simulink model "HRTIM"  (R2023b)
settings: Solver=ode3  StartTime=0.0  StopTime=120e-6  RelTol=1e-3
undefined symbols (not defined in the file): HRTIM_SETB1R_REG_VAL, HRTIM_SETB2R_REG_VAL, HRTIM_SETC1R_REG_VAL, HRTIM_SETC2R_REG_VAL, HRTIM_SL
libraries: dspswit3 x8, simulink x6, simulink_extras x4, hdlsllib x4
(part 1 of 2)
settings Model: Creator=Joe  LastModifiedBy=Joe

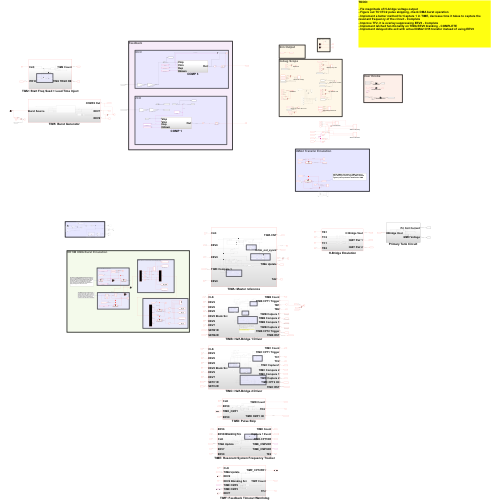
[thumbnail: Simulink's stored preview of the top-level diagram]
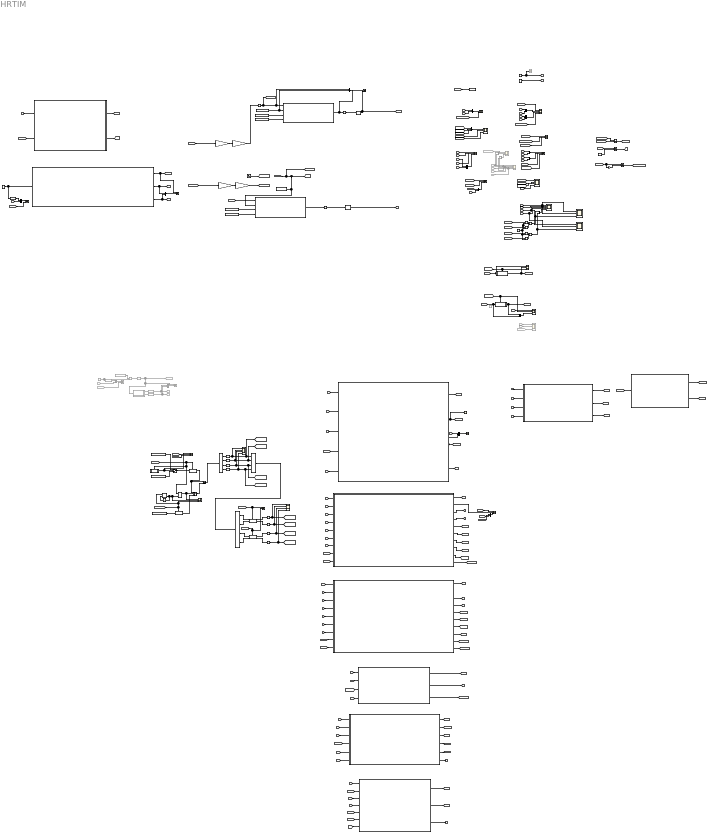
== system HRTIM ==
  note: The DMA2 CH3 trigger is debounced to every 2nd pulse (Hit = 2). This is done so that the output_reset register values can stick for at least 1 resonant cycle, so we are able to witness the pulse skipping waveform at the TB1/2 and TC1/2 outputs
  note: TIMB/C Output 1 and 2 Set Source(s) Shadow Registers
  note: TIMB/C Output 1 and 2 Set Source(s) Active Registers
  note: output_reset DMA Burst Emulation
  note: output_set DMA Burst emulation
  note: Sim Output
  note: ZCD
  note: User Knobs
  note: STM32 System Clocks
  note: Feedback
  note: Debug Scope
  note: HRTIM DMA Burst Emulation
  note: NOTE: DMA2 CH4 write to TIMD Compare 1 goes directly to active register (NOT shadow register) since preload is disabled for TIMD
  note: OCD
  note: TODO:
      |
      | - Fix magnitude of H-bridge voltage output
      | - Figure out TC1/TC2 pulse skipping, check DMA burst operation
      | - Implement a better method for Capture 1 in TIME, decrease time it takes to capture the resonant frequency of the circuit - Complete
      | - Improve TF2, it is overlay suppressing EEV6 - Complete
      | - Implement latched functionality on TIMA EEV9 blanking - COMPLETE
      | - Implement delayed idle exit with actual DMA2 CH5 transfer instead of using EEV9
  note: DMA2 Transfer Emulation
  note: Burst Generator
  note: This seeks to emulate the DMA burst behavior of writing 8 bytes to the HRTIM.BDMADR register when only 4 SFRs are enabled for DMA burst updates (SETB1R,SETB2R, SETC1R and SETC2R). This will update the SFR shadow registers with output_reset[0:3] on 1st DMA2 CH2 trigger, then output_reset[4:7] on 2nd DMA2 CH2. Then resets back to output_reset[0:3] on the 3rd, and on and on.
  APB1 : DiscretePulseGenerator  Period=10  PulseWidth=5  SampleTime=1/(HRTIM_SL.MATLAB.f_discrete)
  APB2 : DiscretePulseGenerator  Period=10  PulseWidth=5  SampleTime=1/(HRTIM_SL.MATLAB.f_discrete)
  COMP 1 : Subsystem
  COMP 3 : Subsystem
  COMP1 : RelationalOperator  Commented=on  Operator=<=  OutDataTypeStr=boolean  RndMeth=Simplest  InputSameDT=off
  COMP3 Hysterisis Lower : Constant  Value=HRTIM_SL.STM32.COMPx_Hdown
  COMP3 Hysterisis Upper : Constant  Value=HRTIM_SL.STM32.COMPx_Hup
  COMP3 INN : Constant  Value=HRTIM_SL.RES_DRV.COMP3.INN
  CT DC Bias : Constant  Value=HRTIM_SL.DRSSTC.vcc/2
  Constant1 : Constant  Value=0  OutDataTypeStr=uint32
  Constant4 : Constant  Commented=on  Value=HRTIM_SL.STM32.VREFINT
  Counter : dspswit3/Counter  Direction=Up  CountEvent=Rising edge  CounterSize=User defined  MaxCount=255  InitialCount=0  Output=Count and Hit  HitValue=HRTIM_SL.MATLAB.output_set_dbnc_cnt  ResetInput=on  SamplesPerFrame=1  Ts=1  CntDtype=double  HitDtype=Boolean
  DMA2 CH1 : Subsystem  TreatAsAtomicUnit=on
  DMA2 CH4 : Subsystem  TreatAsAtomicUnit=on
  Data Type Conversion : DataTypeConversion  OutDataTypeStr=boolean  SaturateOnIntegerOverflow=off  RndMeth=Floor
  Data Type Conversion3 : DataTypeConversion  Commented=on  OutDataTypeStr=boolean  SaturateOnIntegerOverflow=off  RndMeth=Floor
  Data Type Conversion8 : DataTypeConversion  Commented=on  OutDataTypeStr=boolean  SaturateOnIntegerOverflow=off  RndMeth=Floor
  Data Type Conversion9 : DataTypeConversion  Commented=on  OutDataTypeStr=boolean  SaturateOnIntegerOverflow=off  RndMeth=Floor
  Demux : Demux
  Demux1 : Demux
  Disable OCD : Constant  Value=false
  EEV2/6 v FB : Scope  NumInputPorts=2
  FBR : Abs  SaturateOnIntegerOverflow=off
  From1 : From  Commented=on  GotoTag=ZCD_CT_OUT_UNBIASED
  From102 : From  Commented=on  GotoTag=EEV6
  From103 : From  Commented=on  GotoTag=ZCD_CT_OUT
  From20 : From  Commented=on  GotoTag=TB1
  From21 : From  Commented=on  GotoTag=TB2
  From22 : From  Commented=on  GotoTag=TC1
  From23 : From  Commented=on  GotoTag=TC2
  From32 : From  Commented=on  GotoTag=TD2
  From33 : From  Commented=on  GotoTag=EEV8
  From44 : From  Commented=on  GotoTag=DMA2_CH4_TRIGGER
  Goto62 : Goto  Commented=on  GotoTag=EEV7
  Goto63 : Goto  Commented=on  GotoTag=EEV9
  Goto64 : Goto  Commented=on  GotoTag=BURST_SRC
  H-Bridge Emulation : Subsystem
  HBridge v Pri Current v Burst v OCD : Scope  NumInputPorts=3
  HBridge v Txy v FB : Scope  NumInputPorts=4
  HRTIM DMA Burst Op Emulation : Subsystem  TreatAsAtomicUnit=on
  HRTIM DMA Burst Op Emulation1 : Subsystem  TreatAsAtomicUnit=on
  HRTIM EEVx : Scope  NumInputPorts=4
  Half/Full Bridge V OCD Event : Scope  NumInputPorts=4
  Hysterisis Lower : Constant  Value=HRTIM_SL.STM32.COMPx_Hdown
  Hysterisis Upper : Constant  Value=HRTIM_SL.STM32.COMPx_Hup
  Invert ZCD FB : Gain  Gain=-1
  Memory : Memory  Commented=on  InheritSampleTime=on
  Memory2 : Memory  InitialCondition=HRTIM_SETB1R_REG_VAL  InheritSampleTime=on
  Memory3 : Memory  InitialCondition=HRTIM_SETB2R_REG_VAL  InheritSampleTime=on
  Memory4 : Memory  InitialCondition=HRTIM_SETC1R_REG_VAL  InheritSampleTime=on
  Memory5 : Memory  InitialCondition=HRTIM_SETC2R_REG_VAL  InheritSampleTime=on
  Memory6 : Memory  InitialCondition=HRTIM_SETB1R_REG_VAL  InheritSampleTime=on
  Memory7 : Memory  InitialCondition=HRTIM_SETB2R_REG_VAL  InheritSampleTime=on
  Memory8 : Memory  InitialCondition=HRTIM_SETC1R_REG_VAL  InheritSampleTime=on
  Memory9 : Memory  InitialCondition=HRTIM_SETC2R_REG_VAL  InheritSampleTime=on
  Mux{,4,12..13} (4 alike) : Mux  Commented=on  Inputs=2
  Mux{1..3,5..11,14..16,19} (14 alike) : Mux  Inputs=2
  Mux17 : Mux
  Mux18 : Mux  Inputs=3
  OCD Burden Resistor : Gain  Gain=HRTIM_SL.DRSSTC.R_ocd_burden
  OCD CT : Gain  Gain=1/HRTIM_SL.DRSSTC.OCD_CT_N
  OCD Enable/Disable : ManualSwitch
  OR1 : Logic  Operator=OR  IconShape=distinctive  AllPortsSameDT=off  OutDataTypeStr=boolean
  OR3 : Logic  Operator=OR  IconShape=distinctive  AllPortsSameDT=off  OutDataTypeStr=boolean
  Primary Current v Feedback : Scope  NumInputPorts=3
  Primary Tank Circuit : Subsystem
  Pulse Skip Debug : Scope  NumInputPorts=5
  Relational Operator{,1..3} (4 alike) : RelationalOperator  Operator===  OutDataTypeStr=boolean  RndMeth=Simplest  InputSameDT=off
  Rising Edge Of OCB : simulink/Logic and Bit Operations/Detect Rise Positive  vinit=0  OutDataTypeStr=boolean
  Rising Edge Of ZCD FB : simulink/Logic and Bit Operations/Detect Rise Positive  vinit=0  OutDataTypeStr=boolean
  S-R Flip-Flop7 : simulink_extras/Flip Flops/S-R Flip-Flop  initial_condition=0
  SR FF Bypass : ManualSwitch  CurrentSetting=0
  Scope : Scope  Commented=on
  Scope1 : Scope  Commented=on  NumInputPorts=3
  Scope14 : Scope  Commented=on  NumInputPorts=4
  Scope18 : Scope  NumInputPorts=2
  Scope19 : Scope
  Scope2 : Scope  Commented=on  NumInputPorts=2
  Scope20 : Scope
  Scope21 : Scope  NumInputPorts=2
  Scope{3..4,6,23,28,30} (6 alike) : Scope  NumInputPorts=3
  Scope29 : Scope  NumInputPorts=2
  Scope34 : Scope  NumInputPorts=4
  Scope35 : Scope  Commented=on  NumInputPorts=2
  Scope5 : Scope  NumInputPorts=4
  Scope7 : Scope  Commented=on  NumInputPorts=3
  Sum : Sum  Inputs=|++
  Switch1 : Switch  Criteria=u2 ~= 0  SaturateOnIntegerOverflow=off  InputSameDT=off
  Switch2 : Switch  Criteria=u2 ~= 0  SaturateOnIntegerOverflow=off  InputSameDT=off
  TIM2: Start Freq Seed + Lead Time Inject : Subsystem
  TIM5 Burst Gen : DiscretePulseGenerator  Amplitude=HRTIM_SL.DRSSTC.vcc  Period=HRTIM_SL.MATLAB.burst_period_n_samp  PulseWidth=HRTIM_SL.MATLAB.burst_pw_n_samp  PhaseDelay=HRTIM_SL.MATLAB.burst_phase_delay  SampleTime=1/(HRTIM_SL.MATLAB.f_discrete)
  TIM5 Burst Gen1 : DiscretePulseGenerator  Commented=on  Amplitude=HRTIM_SL.DRSSTC.vcc  Period=HRTIM_SL.MATLAB.burst_period_n_samp  PulseWidth=HRTIM_SL.MATLAB.burst_pw_n_samp  SampleTime=1/(HRTIM_SL.MATLAB.f_discrete)
  TIM5: Burst Generator : Subsystem
  TIMA: Master reference : Subsystem
  TIMB Pulse Skip Debug : Scope  NumInputPorts=3
  TIMB: Half-Bridge 1 Driver : Subsystem
  TIMC Pulse Skip Debug : Scope  NumInputPorts=3
  TIMC: Half-Bridge 2 Driver : Subsystem
  TIMD: Pulse Skip : Subsystem
  TIME: Resonant System Frequency Tracker : Subsystem
  TIMF: Feedback Timeout Watchdog : Subsystem
  Tank Circuit v Hbridge : Scope  NumInputPorts=3
  To Workspace : ToWorkspace  VariableName=h_bridge_out  SaveFormat=Timeseries  SampleTime=-1
  Txy v Burst Src v FB : Scope  NumInputPorts=4
  Unit Delay : UnitDelay  SampleTime=-1  HasFrameUpgradeWarning=on
  Update TIMB SETBxR Active Registers : Subsystem  TreatAsAtomicUnit=on
  Update TIMB SETCxR Active Registers : Subsystem  TreatAsAtomicUnit=on
  ZCD Burden Resistor : Gain  Gain=HRTIM_SL.DRSSTC.R_zcd_burden
  ZCD CT : Gain  Gain=1/HRTIM_SL.DRSSTC.ZCD_CT_N
  ZCD Current Feedback : Sin  Amplitude=HRTIM_SL.DRSSTC.vcc/2  Frequency=(HRTIM_SL.DRSSTC.f_pri_res*HRTIM_SL.DRSSTC.f_fb_skew)*2*pi  SampleTime=0
  ZCD FB Select : ManualSwitch  CurrentSetting=0
  ZCD Invert FB Select : ManualSwitch  CurrentSetting=0
  Zero-Order Hold : ZeroOrderHold  SampleTime=1/(HRTIM_SL.MATLAB.f_discrete)
  Zero-Order Hold2 : ZeroOrderHold  SampleTime=1/(HRTIM_SL.MATLAB.f_discrete)
  Zero-Order Hold3 : ZeroOrderHold  Commented=on  SampleTime=1/(HRTIM_SL.MATLAB.f_discrete)
  gen_eev7_eev1 : MATLAB Function  Commented=on  TreatAsAtomicUnit=on
  out_reset_toggle : Subsystem  TreatAsAtomicUnit=on
  output_reset[0:3] : Constant  Value=HRTIM_SL.RES_DRV.output_reset03
  output_reset[4:7] : Constant  Value=HRTIM_SL.RES_DRV.output_reset47
  output_set : Constant  Value=HRTIM_SL.RES_DRV.output_set
  wires:
  Sum/1 -> [ZCD_CT_OUT]  "Biased CT Out"
  CT DC Bias/1 -> COMP 1/2(Vinn), Sum/2  "CT DC Bias"
  Zero-Order Hold/1 -> Rising Edge Of ZCD FB/1  "EEV6"
  APB2/1 -> Scope/1, [APB2]  "APB2"
  APB1/1 -> [APB1]  "APB1"
  From20/1 -> Scope14/1, Mux/1  "TB1"
  From21/1 -> Mux/2, Scope14/2  "TB2"
  From22/1 -> Mux4/1, Scope14/3  "TC1"
  From23/1 -> Mux4/2, Scope14/4  "TC2"
  [ZCD_CT_OUT] -> Scope18/2  "ZCD CT Out"
  [EEV6] -> Mux1/2  "EEV6"
  Mux1/1 -> Scope18/1
  TIM5 Burst Gen/1 -> TIM5: Burst Generator/1(Burst Source), Data Type Conversion/1  "Burst Source"
  Data Type Conversion/1 -> Mux1/1  "Burst Source"
  FBR/1 -> [OCD_FB_RECTIFIED], COMP 3/1(Vinp), Mux2/1  "OCD CT Out Rectified"
  COMP 3/1(Out) -> Zero-Order Hold2/1, Scope23/2  "COMP3 Out"
  DMA2 CH4/1(Out1) -> Mux3/1, [TIMD_CMP1DR]  "TIMD Compare 1"
  [DMA2_CH4_TRIGGER] -> DMA2 CH4/Trigger, Scope28/2  "DMA2 CH4 Trigger"
  [TIME_CNT] -> Scope28/1  "TIME Count"
  Mux3/1 -> Scope28/3
  [DMA2_CH1_TRIGGER] -> DMA2 CH1/Trigger, Scope30/3  "DMA2 CH1 Trigger"
  [TIME_CPT1ER] -> Scope30/1, DMA2 CH1/1(In1)  "TIME Capture 1"
  [APB2] -> TIMD: Pulse Skip/1(CLK)
  [EEV8] -> TIMD: Pulse Skip/2(EEV8)
  [TIMD_CMP1DR] -> TIMD: Pulse Skip/3(TIMD_CMP1)
  [EEV9] -> TIMD: Pulse Skip/4(EEV9)
  TIMD: Pulse Skip/1(TIMD Count) -> [TIMD_CNT]
  TIMD: Pulse Skip/2(TD2) -> [TD2]
  [APB2] -> TIMF: Feedback Timeout Watchdog/1(CLK)
  [TIMA_UPDATE] -> TIMF: Feedback Timeout Watchdog/2(TIMA Update)  "TIMA Update"
  [EEV2] -> TIMF: Feedback Timeout Watchdog/3(EEV2)
  [TE2] -> TIMF: Feedback Timeout Watchdog/4(EEV2 Blanking Src)
  [TIME_CMP2ER] -> TIMF: Feedback Timeout Watchdog/5(TIME CMP2)  "TIME CMP2"
  [TIME_CMP3ER] -> TIMF: Feedback Timeout Watchdog/6(TIME CMP3)  "TIME CMP3"
  [EEV7] -> TIMF: Feedback Timeout Watchdog/7(EEV7)
  TIMF: Feedback Timeout Watchdog/1(TIMF_CPT2FR1) -> [TIMF_CPT2FR1]
  TIMF: Feedback Timeout Watchdog/2(TIMF Count) -> [TIMF_CNT]
  TIMF: Feedback Timeout Watchdog/3(TF2) -> [TF2]
  [EEV6] -> TIME: Resonant System Frequency Tracker/1(EEV6)  "EEV6"
  [TF2] -> TIME: Resonant System Frequency Tracker/2(EEV6 Blanking Src)  "TF2"
  [APB2] -> TIME: Resonant System Frequency Tracker/3(CLK)
  [TIMA_UPDATE] -> TIME: Resonant System Frequency Tracker/4(TIMA Update)  "TIMA Update"
  [EEV7] -> TIME: Resonant System Frequency Tracker/5(EEV7)  "EEV7"
  [EEV9] -> TIME: Resonant System Frequency Tracker/6(EEV9)  "EEV9"
  TIME: Resonant System Frequency Tracker/1(TIME Count) -> [TIME_CNT]
  TIME: Resonant System Frequency Tracker/2(Capture 1 Event) -> [DMA2_CH1_TRIGGER]
  TIME: Resonant System Frequency Tracker/3(TIME.CPT1ER) -> [TIME_CPT1ER]
  TIME: Resonant System Frequency Tracker/4(TIME_CMP2ER) -> [TIME_CMP2ER]
  TIME: Resonant System Frequency Tracker/5(TIME_CMP3ER) -> [TIME_CMP3ER]
  TIME: Resonant System Frequency Tracker/6(TE2) -> [TE2]
  From1/1 -> Scope1/1
  Mux/1 -> Scope1/2
  Mux4/1 -> Scope1/3
  [TIMB_CNT] -> Scope4/1  "TIMB CNT"
  Mux5/1 -> Scope4/3
  [TIMB_CPT1BR] -> Mux5/1  "Capture 1 Reg"
  [TIMB_CMP2BR] -> Mux5/2  "Compare 2 Reg"
  Rising Edge Of ZCD FB/1 -> [EEV6]  "EEV6 RE"
  [EEV9] -> Mux6/2  "EEV9 (BURST RE)"
  [EEV7] -> Mux6/1  "EEV7(BURST LL)"
  [EEV2] -> HRTIM EEVx/1  "EEV2 (TRGO RE)"
  [EEV6] -> HRTIM EEVx/2  "EEV6 (ZCD RE)"
  [EEV8] -> HRTIM EEVx/3  "EEV8 (OCD RE)"
  Mux6/1 -> HRTIM EEVx/4
  [APB2] -> TIMB: Half-Bridge 1 Driver/1(CLK)
  [EEV2] -> TIMB: Half-Bridge 1 Driver/2(EEV2)  "EEV2"
  [EEV6] -> TIMB: Half-Bridge 1 Driver/3(EEV6)  "EEV6"
  TIMB: Half-Bridge 1 Driver/1(TIMB Count) -> [TIMB_CNT]
  TIMB: Half-Bridge 1 Driver/2(TIMB CPT1 Trigger) -> Scope4/2
  TIMB: Half-Bridge 1 Driver/3(TB1) -> [TB1]
  TIMB: Half-Bridge 1 Driver/4(TB2) -> [TB2]
  TIMB: Half-Bridge 1 Driver/7(TIMB Compare 1) -> [TIMB_CMP1BR]
  TIMB: Half-Bridge 1 Driver/6(TIMB Compare 2) -> [TIMB_CMP2BR]
  TIMB: Half-Bridge 1 Driver/5(TIMB Catpure 1) -> [TIMB_CPT1BR]
  TIMC: Half-Bridge 2 Driver/5(TIMC Capture1) -> [TIMC_CPT1BR]
  TIMC: Half-Bridge 2 Driver/6(TIMC Compare 2) -> [TIMC_CMP2BR]
  TIMC: Half-Bridge 2 Driver/8(TIMC Capture 2) -> [TIMC_CPT2CR]  "TIMC CPT2 eg"
  TIMC: Half-Bridge 2 Driver/7(TIMC Compare 1) -> [TIMC_CMP1CR]
  TIMC: Half-Bridge 2 Driver/4(TC2) -> [TC2]
  TIMC: Half-Bridge 2 Driver/3(TC1) -> [TC1]
  TIMC: Half-Bridge 2 Driver/1(TIMC Count) -> [TIMC_CNT]
  [APB2] -> TIMC: Half-Bridge 2 Driver/1(CLK)
  [EEV2] -> TIMC: Half-Bridge 2 Driver/2(EEV2)
  [EEV6] -> TIMC: Half-Bridge 2 Driver/3(EEV6)
  [EEV8] -> TIMC: Half-Bridge 2 Driver/4(EEV8)
  [TD2] -> TIMC: Half-Bridge 2 Driver/5(EEV8 Blank Src)
  TIMC: Half-Bridge 2 Driver/9(TIMC CPT2 Hit) -> [DMA2_CH4_TRIGGER]  "TIMC CPT2 Hit"
  Rising Edge Of OCB/1 -> [EEV8_RE], Scope23/3  "EEV8 RE"
  TIMB: Half-Bridge 1 Driver/8(TIMB Capture 2) -> [TIMB_CPT2BR]
  TIMB: Half-Bridge 1 Driver/9(TIMB CPT2 Trigger) -> [DMA2_CH2_TRIGGER]  "TIMB CPT2 Trigger"
  [EEV8] -> TIMB: Half-Bridge 1 Driver/4(EEV8)  "EEV8"
  [TA2] -> TIMB: Half-Bridge 1 Driver/5(EEV8 Blank Src)
  [APB2] -> TIMA: Master reference/1(CLK)
  [EEV6] -> TIMA: Master reference/2(EEV6)  "EEV6"
  [EEV9] -> TIMA: Master reference/3(EEV9)  "EEV9"
  [TIMD_CMP1DR] -> TIMA: Master reference/4(TIMD Compare 1)  "TIMD Compare 1"
  [EEV8] -> TIMA: Master reference/5(EEV8)  "EEV8"
  TIMA: Master reference/1(TIMA CNT) -> [TIMA_CNT]
  TIMA: Master reference/2(hrtim_out_sync2) -> Scope19/1, [hrtim_out_sync2]  "hrtim_out_sync2"
  TIMA: Master reference/3(TIMA Update) -> Mux7/2, [TIMA_UPDATE]  "TIMA Update"
  TIMA: Master reference/4(TA2) -> [TA2]
  Mux7/1 -> Scope20/1
  [EEV6] -> Mux7/1
  Mux8/1 -> Scope21/2
  [EEV7] -> TIMB: Half-Bridge 1 Driver/7(EEV7)
  [EEV9] -> TIMB: Half-Bridge 1 Driver/6(EEV9)
  [TB1] -> Mux10/1  "TB1"
  [TB2] -> Mux10/2  "TB2"
  [TC2] -> Mux11/2  "TC2"
  [TC1] -> Mux11/1  "TC1"
  Mux10/1 -> Txy v Burst Src v FB/1
  Mux11/1 -> Txy v Burst Src v FB/2
  [BURST_SRC] -> Txy v Burst Src v FB/3  "Burst Src"
  [ZCD_CT_OUT_UNBIASED] -> Txy v Burst Src v FB/4  "ZCD"
  [EEV7] -> TIMC: Half-Bridge 2 Driver/7(EEV7)
  [EEV9] -> TIMC: Half-Bridge 2 Driver/6(EEV9)
  Switch1/1 -> HRTIM DMA Burst Op Emulation/1(In1)
  [DMA2_CH2_TRIGGER] -> out_reset_toggle/Trigger, S-R Flip-Flop7/1, HRTIM DMA Burst Op Emulation/Trigger  "TIMB Capture 2"
  output_reset[0:3]/1 -> Switch1/1
  output_reset[4:7]/1 -> Switch1/3
  Demux/3 -> Memory8/1
  Demux/4 -> Memory9/1
  HRTIM DMA Burst Op Emulation/1(Out1) -> SR FF Bypass/1, Switch2/1  "SETxyR Shadow Registers"
  ZCD CT/1 -> ZCD Burden Resistor/1
  [ZCD_FB_SRC] -> [ZCD_CT_OUT_UNBIASED], Sum/1  "ZCD Out"
  DMA2 CH1/1(Out1) -> Scope30/2, [TIM2_ARR_SH]  "TIM2 ARR Shadow Register"
  [ZCD_CT_OUT] -> COMP 1/1(Vinp)  "Vinp"
  Hysterisis Upper/1 -> COMP 1/3(Hup)  "Hup"
  Hysterisis Lower/1 -> COMP 1/4(Hdown)  "Hdown"
  COMP 1/1(Out) -> Zero-Order Hold/1  "COMP1 Out"
  ZCD Burden Resistor/1 -> [ZCD_FB_SRC_SAMPLED]  "Sampled Feedback"
  ZCD Current Feedback/1 -> [ZCD_FB_SRC_GENERATED]  "Generated Feedback"
  ZCD FB Select/1 -> [ZCD_FB_SRC]  "ZCD Out"
  [ZCD_FB_SRC_GENERATED] -> ZCD FB Select/1
  [ZCD_FB_SRC_SAMPLED] -> ZCD FB Select/2
  COMP3 Hysterisis Upper/1 -> COMP 3/3(Hup)  "Hup"
  COMP3 Hysterisis Lower/1 -> COMP 3/4(Hdown)  "Hdown"
  COMP3 INN/1 -> Mux2/2, COMP 3/2(Vinn)  "COMP3 INN"
  Zero-Order Hold2/1 -> Rising Edge Of OCB/1  "EEV8"
  Mux2/1 -> Scope23/1
  OCD CT/1 -> OCD Burden Resistor/1
  OCD Burden Resistor/1 -> FBR/1  "Sampled Feedback"
  [HBRIDGE_OUT] -> To Workspace/1
  Disable OCD/1 -> OCD Enable/Disable/2
  OCD Enable/Disable/1 -> [EEV8]  "EEV8"
  [EEV8_RE] -> OCD Enable/Disable/1  "EEV8 Rising Edge"
  [PRI_CURRENT] -> Primary Current v Feedback/1  "Primary Current"
  [ZCD_CT_OUT_UNBIASED] -> Primary Current v Feedback/2  "ZCD FB"
  [OCD_FB_RECTIFIED] -> Primary Current v Feedback/3  "OCD FB RECT"
  [TB2] -> Mux14/2  "TB2"
  [TC2] -> Mux15/2  "TC2"
  Mux15/1 -> HBridge v Txy v FB/3
  [TC1] -> Mux15/1  "TC1"
  [TB1] -> Mux14/1  "TB1"
  Mux14/1 -> HBridge v Txy v FB/2
  [ZCD_CT_OUT_UNBIASED] -> HBridge v Txy v FB/4  "ZCD"
  [HBRIDGE_OUT] -> HBridge v Txy v FB/1  "H Bridge Out"
  [TIME_CPT1ER] -> DMA2 CH4/1(In1), Mux3/2  "TIME Capture 1"
  gen_eev7_eev1/2(eev9) -> Data Type Conversion9/1
  Data Type Conversion9/1 -> Goto63/1, Mux13/2  "EEV9"
  Mux13/1 -> Scope35/2
  Zero-Order Hold3/1 -> Goto64/1, gen_eev7_eev1/1(comp4_out), Scope35/1  "COMP4 Out"
  From102/1 -> Mux12/2  "EEV6"
  Constant4/1 -> COMP1/1
  gen_eev7_eev1/1(eev7) -> Data Type Conversion8/1
  Mux12/1 -> Scope2/1
  Data Type Conversion8/1 -> Mux13/1, Goto62/1  "EEV7"
  Data Type Conversion3/1 -> Mux12/1  "Burst Source"
  TIM5 Burst Gen1/1 -> Data Type Conversion3/1, COMP1/2  "Burst Source"
  COMP1/1 -> Zero-Order Hold3/1
  From103/1 -> Scope2/2  "ZCD CT Out"
  [EEV2] -> Mux16/1  "EEV2 (TRGO RE)"
  [EEV6] -> Mux16/2  "EEV6 (ZCD RE)"
  Mux16/1 -> EEV2/6 v FB/1
  [ZCD_CT_OUT_UNBIASED] -> EEV2/6 v FB/2  "ZCD"
  [ZCD_PRI_CURRENT] -> ZCD CT/1
  [PRI_CURRENT] -> ZCD Invert FB Select/1, Invert ZCD FB/1  "Primary Current"
  Invert ZCD FB/1 -> ZCD Invert FB Select/2
  [PRI_CURRENT] -> OCD CT/1  "Primary Current"
  ZCD Invert FB Select/1 -> [ZCD_PRI_CURRENT]  "To ZCD Feedback Circuit"
  [PRI_CURRENT] -> Tank Circuit v Hbridge/2  "Pri Current"
  [MMC_Voltage] -> Tank Circuit v Hbridge/3  "MMC Voltage"
  [IGBT_PAIR1] -> Mux18/1  "IGBT Pair1"
  Mux18/1 -> Tank Circuit v Hbridge/1
  [IGBT_PAIR2] -> Mux18/2  "IGBT Pair2"
  [HBRIDGE_OUT] -> Mux18/3  "Hbridge Out"
  [APB1] -> TIM2: Start Freq Seed + Lead Time Inject/1(CLK)  "APB1"
  [hrtim_out_sync2] -> TIM2: Start Freq Seed + Lead Time Inject/2(ITR10)  "ITR10"
  TIM2: Start Freq Seed + Lead Time Inject/1(TIM2 Count) -> [TIM2_CNT]  "TIM2 CNT"
  TIM2: Start Freq Seed + Lead Time Inject/2(TIM2 TRGO RE) -> [EEV2]  "TIM2 TRGO RE"
  out_reset_toggle/1(Out1) -> Scope6/1, Switch1/2  "out_reset_toggle"
  Demux1/1 -> Update TIMB SETBxR Active Registers/1(In1)  "SETB1R SH"
  Update TIMB SETBxR Active Registers/1(Out1) -> Memory2/1
  Demux1/2 -> Update TIMB SETBxR Active Registers/2(In2)  "SETB2R SH"
  Update TIMB SETBxR Active Registers/2(Out2) -> Memory3/1  "SETB2R Active"
  [TIMB_UPDATE_TRIG] -> Scope29/1, Update TIMB SETBxR Active Registers/Trigger  "TIMB Update Trigger"
  Demux1/3 -> Update TIMB SETCxR Active Registers/1(In1)  "SETC1R SH"
  Demux1/4 -> Update TIMB SETCxR Active Registers/2(In2)  "SETC2R SH"
  Update TIMB SETCxR Active Registers/1(Out1) -> Memory4/1  "SETC1R Active"
  Update TIMB SETCxR Active Registers/2(Out2) -> Memory5/1  "SETC2R Active"
  [TIMC_UPDATE_TRIG] -> Scope29/2, Update TIMB SETCxR Active Registers/Trigger  "TIMC Update Trigger"
  TIMB: Half-Bridge 1 Driver/10(TIMB RST) -> [TIMB_UPDATE_TRIG]  "TIMB RST Triggers Update"
  TIMC: Half-Bridge 2 Driver/10(TIMC RST) -> [TIMC_UPDATE_TRIG]  "TIMC RST Triggers Update"
  [TIMB_SETB1R] -> TIMB: Half-Bridge 1 Driver/8(SETB1R)
  [TIMB_SETB2R] -> TIMB: Half-Bridge 1 Driver/9(SETB2R)
  [TIMC_SETC2R] -> TIMC: Half-Bridge 2 Driver/9(SETC2R)
  [TIMC_SETC1R] -> TIMC: Half-Bridge 2 Driver/8(SETC1R)
  Memory2/1 -> [TIMB_SETB1R], Scope34/1
  Memory3/1 -> [TIMB_SETB2R], Scope34/2
  Memory4/1 -> Scope34/3, [TIMC_SETC1R]
  Memory5/1 -> Scope34/4, [TIMC_SETC2R]
  Memory6/1 -> Mux17/1, [TIMB_SETB1R_SH], Scope5/1  "SETB1R SH"
  Memory7/1 -> Mux17/2, [TIMB_SETB2R_SH], Scope5/2  "SETB2R SH"
  Memory8/1 -> [TIMC_SETC1R_SH], Mux17/3, Scope5/3  "SETC1R SH"
  Memory9/1 -> [TIMC_SETC2R_SH], Mux17/4, Scope5/4  "SETC2R SH"
  Demux/1 -> Memory6/1
  Demux/2 -> Memory7/1
  Mux17/1 -> Demux1/1
  [BURST_SRC] -> Mux19/1  "Burst Src"
  [EEV8] -> Mux19/2  "EEV8"
  [HBRIDGE_OUT] -> HBridge v Pri Current v Burst v OCD/1  "Hbridge Out"
  [PRI_CURRENT] -> HBridge v Pri Current v Burst v OCD/2  "Pri Current"
  Mux19/1 -> HBridge v Pri Current v Burst v OCD/3
  TIMD: Pulse Skip/3("TIMD CMP1 Hit ") -> [DMA2_CH3_TRIGGER]  "TIMD CMP1 Hit"
  output_set/1 -> HRTIM DMA Burst Op Emulation1/1(In1)
  S-R Flip-Flop7/1 -> Switch2/2, Scope3/1  "Q"
  [DMA2_CH3_TRIGGER] -> Scope3/3, Counter/1, HRTIM DMA Burst Op Emulation1/Trigger  "TIMD Compare 1"
  HRTIM DMA Burst Op Emulation1/1(Out1) -> Switch2/3
  SR FF Bypass/1 -> Demux/1
  Switch2/1 -> SR FF Bypass/2
  Counter/2 -> S-R Flip-Flop7/2, Scope3/2, Unit Delay/1  "SR FF Reset"
  Unit Delay/1 -> Counter/2
  TIM5: Burst Generator/3(EEV9) -> [EEV9], Mux8/2  "EEV9"
  TIM5: Burst Generator/2(EEV7) -> Mux8/1, [EEV7]  "EEV7"
  TIM5: Burst Generator/1(COMP4 Out) -> Scope21/1, [BURST_SRC]
  Relational Operator/1 -> OR3/1
  [TIMB_SETB1R] -> Relational Operator/1
  Relational Operator1/1 -> OR3/2
  Constant1/1 -> Relational Operator1/2, Relational Operator/2, Relational Operator2/2, Relational Operator3/2
  [TIMB_SETB2R] -> Relational Operator1/1
  [TIMC_SETC2R] -> Relational Operator3/1
  Relational Operator2/1 -> OR1/1
  Relational Operator3/1 -> OR1/2
  [TIMC_SETC1R] -> Relational Operator2/1
  [TB1] -> Pulse Skip Debug/1, TIMB Pulse Skip Debug/1  "TB1"
  [TB2] -> Pulse Skip Debug/2, TIMB Pulse Skip Debug/2  "TB2"
  [TC1] -> TIMC Pulse Skip Debug/1, Pulse Skip Debug/3  "TC1"
  OR3/1 -> Mux9/1, TIMB Pulse Skip Debug/3  "TIMB SET Disabled"
  OR1/1 -> TIMC Pulse Skip Debug/3, Mux9/2  "TIMC SET Disabled"
  [TC2] -> Pulse Skip Debug/4, TIMC Pulse Skip Debug/2  "TC2"
  Mux9/1 -> Pulse Skip Debug/5
  [TIMB_UPDATE_TRIG] -> Scope6/2  "TIMB Update Trigger"
  [TIMC_UPDATE_TRIG] -> Scope6/3  "TIMC Update Trigger"
  From32/1 -> Scope7/1  "TD2"
  From33/1 -> Scope7/2  "EEV8"
  From44/1 -> Scope7/3  "DMA2 CH4 Trigger"
  [IGBT_PAIR1] -> Half/Full Bridge V OCD Event/1  "Half Bridge 1"
  [EEV8] -> Half/Full Bridge V OCD Event/4  "EEV8 (OCD)"
  [HBRIDGE_OUT] -> Half/Full Bridge V OCD Event/3  "Full Bridge"
  [IGBT_PAIR2] -> Half/Full Bridge V OCD Event/2  "Half Bridge 2"
  [TB1] -> H-Bridge Emulation/1(TB1)  "TB1"
  [TC2] -> H-Bridge Emulation/2(TC2)  "TC2"
  [TC1] -> H-Bridge Emulation/3(TC1)  "TC1"
  [TB2] -> H-Bridge Emulation/4(TB2)  "TB2"
  H-Bridge Emulation/1(H Bridge Vout) -> [HBRIDGE_OUT]  "Full Bridge Out"
  H-Bridge Emulation/2(IGBT Pair 1) -> [IGBT_PAIR1]  "Half Bridge 1 Out"
  H-Bridge Emulation/3(IGBT Pair 2) -> [IGBT_PAIR2]  "Half Bridge 2 Out"
  [HBRIDGE_OUT] -> Primary Tank Circuit/1(HBridge Vout)  "HBridge Vout"
  Primary Tank Circuit/1(Pri Coil Current) -> [PRI_CURRENT]  "Primary Current"
  Primary Tank Circuit/2(MMC Voltage) -> [MMC_Voltage]  "MMC Voltage"

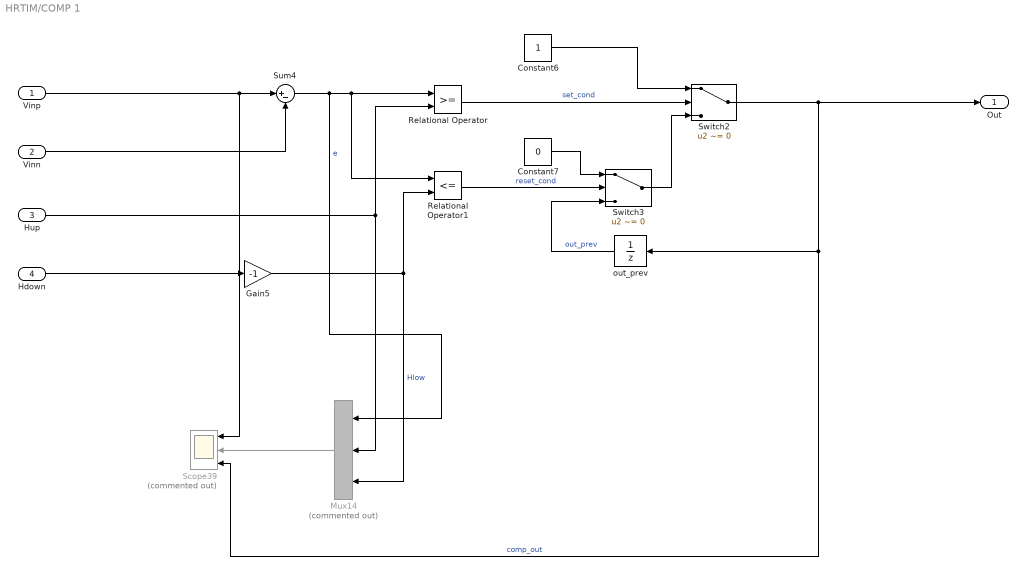
== system HRTIM/COMP 1 ==
  Vinp : Inport
  Vinn : Inport  Port=2
  Hup : Inport  Port=3
  Hdown : Inport  Port=4
  Constant6 : Constant
  Constant7 : Constant  Value=0
  Gain5 : Gain  Gain=-1
  Mux14 : Mux  Commented=on  Inputs=3
  Relational Operator : RelationalOperator  OutDataTypeStr=boolean  RndMeth=Simplest  InputSameDT=off
  Relational Operator1 : RelationalOperator  Operator=<=  OutDataTypeStr=boolean  RndMeth=Simplest  InputSameDT=off
  Scope39 : Scope  Commented=on  NumInputPorts=3
  Sum4 : Sum  Inputs=|+-
  Switch2 : Switch  Criteria=u2 ~= 0  SaturateOnIntegerOverflow=off  InputSameDT=off
  Switch3 : Switch  Criteria=u2 ~= 0  SaturateOnIntegerOverflow=off  InputSameDT=off
  out_prev : UnitDelay  SampleTime=-1  HasFrameUpgradeWarning=on
  Out : Outport
  wires:
  Sum4/1 -> Mux14/1, Relational Operator/1, Relational Operator1/1  "e"
  Relational Operator/1 -> Switch2/2  "set_cond"
  Switch2/1 -> Out/1, out_prev/1, Scope39/3  "comp_out"
  Relational Operator1/1 -> Switch3/2  "reset_cond"
  Mux14/1 -> Scope39/2
  Vinn/1 -> Sum4/2
  Gain5/1 -> Mux14/3, Relational Operator1/2  "Hlow"
  Constant6/1 -> Switch2/1
  out_prev/1 -> Switch3/3  "out_prev"
  Hup/1 -> Mux14/2, Relational Operator/2
  Constant7/1 -> Switch3/1
  Vinp/1 -> Scope39/1, Sum4/1
  Switch3/1 -> Switch2/3
  Hdown/1 -> Gain5/1

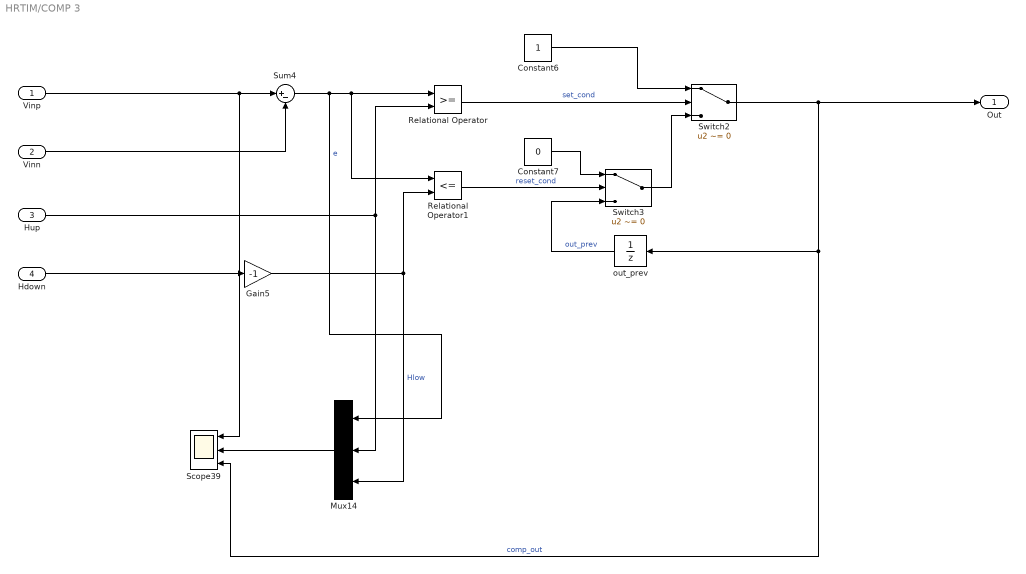
== system HRTIM/COMP 3 ==
  Vinp : Inport
  Vinn : Inport  Port=2
  Hup : Inport  Port=3
  Hdown : Inport  Port=4
  Constant6 : Constant
  Constant7 : Constant  Value=0
  Gain5 : Gain  Gain=-1
  Mux14 : Mux  Inputs=3
  Relational Operator : RelationalOperator  OutDataTypeStr=boolean  RndMeth=Simplest  InputSameDT=off
  Relational Operator1 : RelationalOperator  Operator=<=  OutDataTypeStr=boolean  RndMeth=Simplest  InputSameDT=off
  Scope39 : Scope  NumInputPorts=3
  Sum4 : Sum  Inputs=|+-
  Switch2 : Switch  Criteria=u2 ~= 0  SaturateOnIntegerOverflow=off  InputSameDT=off
  Switch3 : Switch  Criteria=u2 ~= 0  SaturateOnIntegerOverflow=off  InputSameDT=off
  out_prev : UnitDelay  SampleTime=-1  HasFrameUpgradeWarning=on
  Out : Outport
  wires:
  Sum4/1 -> Mux14/1, Relational Operator/1, Relational Operator1/1  "e"
  Relational Operator/1 -> Switch2/2  "set_cond"
  Switch2/1 -> Out/1, out_prev/1, Scope39/3  "comp_out"
  Relational Operator1/1 -> Switch3/2  "reset_cond"
  Mux14/1 -> Scope39/2
  Vinn/1 -> Sum4/2
  Gain5/1 -> Mux14/3, Relational Operator1/2  "Hlow"
  Constant6/1 -> Switch2/1
  out_prev/1 -> Switch3/3  "out_prev"
  Hup/1 -> Mux14/2, Relational Operator/2
  Constant7/1 -> Switch3/1
  Vinp/1 -> Scope39/1, Sum4/1
  Switch3/1 -> Switch2/3
  Hdown/1 -> Gain5/1

== system HRTIM/DMA2 CH1 ==
  In1 : Inport
  Trigger : TriggerPort  VariantControl=(inherit)
  Out1 : Outport
  wires:
  In1/1 -> Out1/1

== system HRTIM/DMA2 CH4 ==
  In1 : Inport
  Trigger : TriggerPort  VariantControl=(inherit)
  Out1 : Outport
  wires:
  In1/1 -> Out1/1

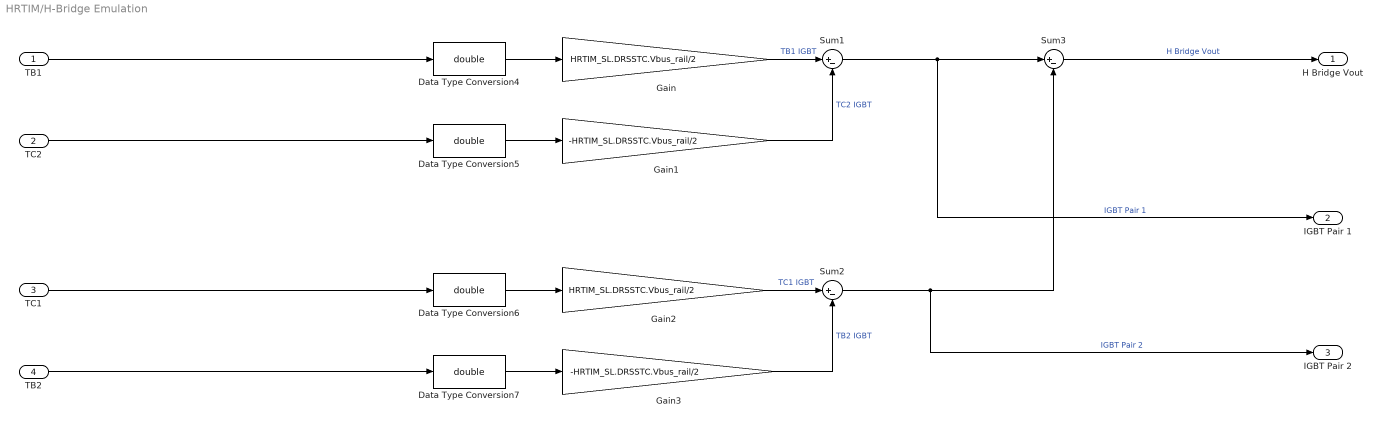
== system HRTIM/H-Bridge Emulation ==
  TB1 : Inport
  TC2 : Inport  Port=2
  TC1 : Inport  Port=3
  TB2 : Inport  Port=4
  Data Type Conversion{4..7} (4 alike) : DataTypeConversion  OutDataTypeStr=double  SaturateOnIntegerOverflow=off  RndMeth=Floor
  Gain : Gain  Gain=HRTIM_SL.DRSSTC.Vbus_rail/2
  Gain1 : Gain  Gain=-HRTIM_SL.DRSSTC.Vbus_rail/2
  Gain2 : Gain  Gain=HRTIM_SL.DRSSTC.Vbus_rail/2
  Gain3 : Gain  Gain=-HRTIM_SL.DRSSTC.Vbus_rail/2
  Sum1 : Sum  Inputs=|+-
  Sum2 : Sum  Inputs=|+-
  Sum3 : Sum  Inputs=|+-
  H Bridge Vout : Outport
  IGBT Pair 1 : Outport  Port=2
  IGBT Pair 2 : Outport  Port=3
  wires:
  Gain2/1 -> Sum2/1  "TC1 IGBT"
  Sum1/1 -> IGBT Pair 1/1, Sum3/1  "IGBT Pair 1"
  Data Type Conversion7/1 -> Gain3/1
  Gain1/1 -> Sum1/2  "TC2 IGBT"
  Data Type Conversion4/1 -> Gain/1
  Sum2/1 -> IGBT Pair 2/1, Sum3/2  "IGBT Pair 2"
  Data Type Conversion6/1 -> Gain2/1
  Gain3/1 -> Sum2/2  "TB2 IGBT"
  Gain/1 -> Sum1/1  "TB1 IGBT"
  Data Type Conversion5/1 -> Gain1/1
  TB1/1 -> Data Type Conversion4/1
  TC1/1 -> Data Type Conversion6/1
  Sum3/1 -> H Bridge Vout/1  "H Bridge Vout"
  TB2/1 -> Data Type Conversion7/1
  TC2/1 -> Data Type Conversion5/1

== system HRTIM/HRTIM DMA Burst Op Emulation ==
  In1 : Inport
  Trigger : TriggerPort  VariantControl=(inherit)
  Out1 : Outport  InitialOutput=HRTIM_SL.RES_DRV.output_set
  wires:
  In1/1 -> Out1/1

== system HRTIM/HRTIM DMA Burst Op Emulation1 ==
  In1 : Inport
  Trigger : TriggerPort  VariantControl=(inherit)
  Out1 : Outport  InitialOutput=HRTIM_SL.RES_DRV.output_set
  wires:
  In1/1 -> Out1/1

== system HRTIM/Primary Tank Circuit ==
  HBridge Vout : Inport
  Demux2 : Demux  Outputs=2
  Primary Tank Circuit : StateSpace  A=HRTIM_SL.MATLAB.PRI_TANK.A  B=HRTIM_SL.MATLAB.PRI_TANK.B  C=HRTIM_SL.MATLAB.PRI_TANK.C  D=HRTIM_SL.MATLAB.PRI_TANK.D  InitialCondition=HRTIM_SL.MATLAB.PRI_TANK.x0
  Scope36 : Scope  Commented=on  NumInputPorts=3
  Pri Coil Current : Outport
  MMC Voltage : Outport  Port=2
  wires:
  Demux2/1 -> Pri Coil Current/1, Scope36/2  "Pri Coil Current"
  HBridge Vout/1 -> Primary Tank Circuit/1, Scope36/1
  Primary Tank Circuit/1 -> Demux2/1
  Demux2/2 -> MMC Voltage/1, Scope36/3  "MMC Voltage"

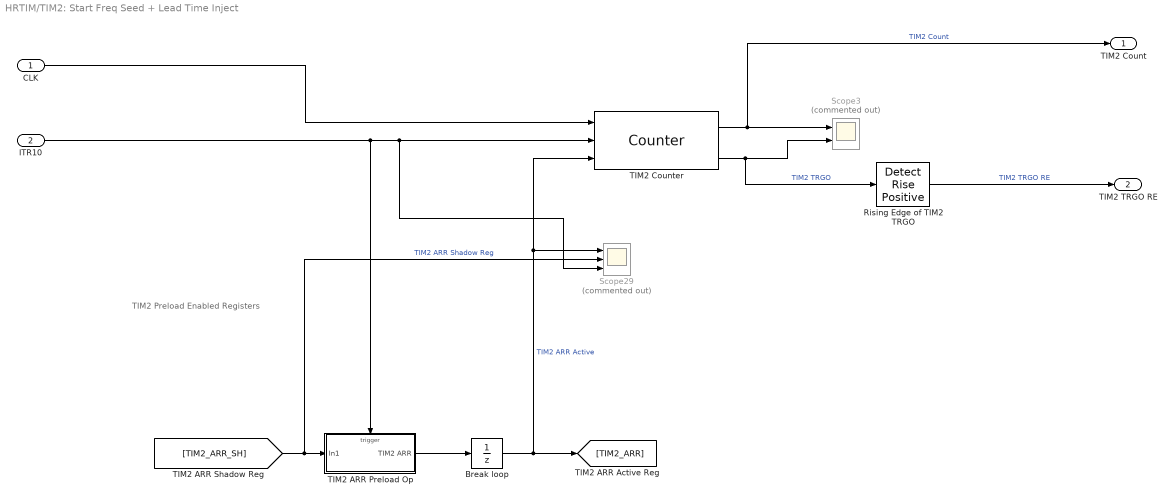
== system HRTIM/TIM2: Start Freq Seed + Lead Time Inject ==
  note: TIM2 Preload Enabled Registers
  CLK : Inport
  ITR10 : Inport  Port=2
  Break loop : UnitDelay  InitialCondition=HRTIM_SL.RES_DRV.TIM2.ARR  SampleTime=-1  HasFrameUpgradeWarning=on
  Rising Edge of TIM2 TRGO : simulink/Logic and Bit Operations/Detect Rise Positive  vinit=0  OutDataTypeStr=boolean
  Scope29 : Scope  Commented=on  NumInputPorts=3
  Scope3 : Scope  Commented=on  NumInputPorts=2
  TIM2 ARR Preload Op : Subsystem  TreatAsAtomicUnit=on
  TIM2 Counter : dspswit3/Counter  Direction=Down  CountEvent=Rising edge  CounterSize=Specify via input port  MaxCount=HRTIM_SL.TIM2.ARR  InitialCount=0  Output=Count and Hit  HitValue=HRTIM_SL.RES_DRV.TIM2.CCR1  ResetInput=on  SamplesPerFrame=1  Ts=1  CntDtype=uint16  HitDtype=Logical
  TIM2 Count : Outport
  TIM2 TRGO RE : Outport  Port=2
  wires:
  CLK/1 -> TIM2 Counter/1
  [TIM2_ARR_SH] -> TIM2 ARR Preload Op/1(In1), Scope29/2  "TIM2 ARR Shadow Reg"
  TIM2 Counter/1 -> TIM2 Count/1, Scope3/1  "TIM2 Count"
  ITR10/1 -> TIM2 ARR Preload Op/Trigger, TIM2 Counter/2, Scope29/3
  TIM2 ARR Preload Op/1(TIM2 ARR) -> Break loop/1
  Break loop/1 -> [TIM2_ARR], TIM2 Counter/3, Scope29/1  "TIM2 ARR Active"
  TIM2 Counter/2 -> Rising Edge of TIM2 TRGO/1, Scope3/2  "TIM2 TRGO"
  Rising Edge of TIM2 TRGO/1 -> TIM2 TRGO RE/1  "TIM2 TRGO RE"

== system HRTIM/TIM5: Burst Generator ==
  Burst Source : Inport
  COMP 4 : Subsystem
  COMP4 Hysterisis Lower : Constant  Value=HRTIM_SL.STM32.COMPx_Hdown
  COMP4 Hysterisis Upper : Constant  Value=HRTIM_SL.STM32.COMPx_Hup
  Data Type Conversion1 : DataTypeConversion  OutDataTypeStr=boolean  SaturateOnIntegerOverflow=off  RndMeth=Floor
  Data Type Conversion2 : DataTypeConversion  OutDataTypeStr=boolean  SaturateOnIntegerOverflow=off  RndMeth=Floor
  STM32 Internal Reference : Constant  Value=HRTIM_SL.STM32.VREFINT
  Zero-Order Hold1 : ZeroOrderHold  SampleTime=1/(HRTIM_SL.MATLAB.f_discrete)
  gen_eev7_eev9 : MATLAB Function  TreatAsAtomicUnit=on
  COMP4 Out : Outport
  EEV7 : Outport  Port=2
  EEV9 : Outport  Port=3
  wires:
  COMP4 Hysterisis Upper/1 -> COMP 4/3(Hup)  "Hup"
  Zero-Order Hold1/1 -> COMP4 Out/1, gen_eev7_eev9/1(comp4_out)  "COMP4 Out"
  gen_eev7_eev9/2(eev9) -> Data Type Conversion2/1
  COMP4 Hysterisis Lower/1 -> COMP 4/4(Hdown)  "Hdown"
  gen_eev7_eev9/1(eev7) -> Data Type Conversion1/1
  STM32 Internal Reference/1 -> COMP 4/2(Vinn)  "Vinn"
  COMP 4/1(Out) -> Zero-Order Hold1/1  "COMP4 Output"
  Burst Source/1 -> COMP 4/1(Vinp)
  Data Type Conversion1/1 -> EEV7/1  "EEV7"
  Data Type Conversion2/1 -> EEV9/1  "EEV9"

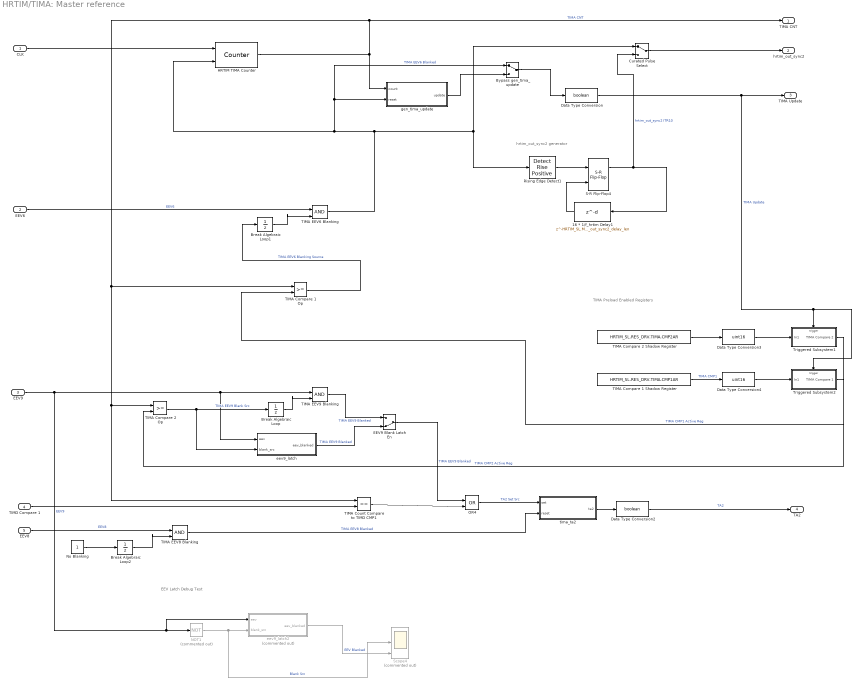
== system HRTIM/TIMA: Master reference ==
  note: EEV Latch Debug Test
  note: hrtim_out_sync2 generator
  note: TIMA Preload Enabled Registers
  CLK : Inport
  EEV6 : Inport  Port=2
  EEV9 : Inport  Port=3
  TIMD Compare 1 : Inport  Port=4
  EEV8 : Inport  Port=5
  16 * 1/f_hrtim Delay1 : Delay  DelayLength=HRTIM_SL.MATLAB.hrtim_out_sync2_delay_len  InitialCondition=0  UseCircularBuffer=on
  Break Algebraic Loop : UnitDelay  SampleTime=-1  HasFrameUpgradeWarning=on
  Break Algebraic Loop1 : UnitDelay  SampleTime=-1  HasFrameUpgradeWarning=on
  Break Algebraic Loop2 : UnitDelay  SampleTime=-1  HasFrameUpgradeWarning=on
  Bypass gen_tima_update : ManualSwitch
  Curated Pulse Select : ManualSwitch
  Data Type Conversion : DataTypeConversion  OutDataTypeStr=boolean  SaturateOnIntegerOverflow=off  RndMeth=Floor
  Data Type Conversion2 : DataTypeConversion  OutDataTypeStr=boolean  SaturateOnIntegerOverflow=off  RndMeth=Floor
  Data Type Conversion3 : DataTypeConversion  OutDataTypeStr=uint16  SaturateOnIntegerOverflow=off  RndMeth=Floor
  Data Type Conversion4 : DataTypeConversion  OutDataTypeStr=uint16  SaturateOnIntegerOverflow=off  RndMeth=Floor
  EEV9 Blank Latch En : ManualSwitch  CurrentSetting=0
  HRTIM TIMA Counter : dspswit3/Counter  Direction=Up  CountEvent=Rising edge  CounterSize=16 bits  MaxCount=HRTIM_SL.HRTIM_TIMx_FS  InitialCount=0  Output=Count  HitValue=32  ResetInput=on  SamplesPerFrame=1  Ts=1  CntDtype=uint16  HitDtype=Logical
  NOT1 : Logic  Commented=on  Operator=NOT  IconShape=distinctive  AllPortsSameDT=off  OutDataTypeStr=boolean
  No Blanking : Constant
  OR4 : Logic  Operator=OR  IconShape=distinctive  AllPortsSameDT=off  OutDataTypeStr=boolean
  Rising Edge Detect1 : simulink/Logic and Bit Operations/Detect Rise Positive  vinit=0  OutDataTypeStr=boolean
  S-R Flip-Flop4 : simulink_extras/Flip Flops/S-R Flip-Flop  initial_condition=0
  Scope4 : Scope  Commented=on  NumInputPorts=3
  TIMA Compare 1 Op : RelationalOperator  OutDataTypeStr=boolean  RndMeth=Simplest  InputSameDT=off
  TIMA Compare 1 Shadow Register : Constant  Value=HRTIM_SL.RES_DRV.TIMA.CMP1AR
  "TIMA Compare 2 Op " : RelationalOperator  OutDataTypeStr=boolean  RndMeth=Simplest  InputSameDT=off
  TIMA Compare 2 Shadow Register : Constant  Value=HRTIM_SL.RES_DRV.TIMA.CMP2AR
  TIMA Count Compare to TIMD CMP1 : RelationalOperator  Operator===  OutDataTypeStr=boolean  RndMeth=Simplest  InputSameDT=off
  TIMA EEV6 Blanking : Logic  IconShape=distinctive  AllPortsSameDT=off  OutDataTypeStr=boolean
  TIMA EEV8 Blanking : Logic  IconShape=distinctive  AllPortsSameDT=off  OutDataTypeStr=boolean
  TIMA EEV9 Blanking : Logic  IconShape=distinctive  AllPortsSameDT=off  OutDataTypeStr=boolean
  Triggered Subsystem1 : Subsystem  TreatAsAtomicUnit=on
  Triggered Subsystem2 : Subsystem  TreatAsAtomicUnit=on
  eev9_latch : MATLAB Function  TreatAsAtomicUnit=on
  eev9_latch2 : MATLAB Function  Commented=on  TreatAsAtomicUnit=on
  gen_tima_update : MATLAB Function  TreatAsAtomicUnit=on
  tima_ta2 : MATLAB Function  TreatAsAtomicUnit=on
  TIMA CNT : Outport
  hrtim_out_sync2 : Outport  Port=2
  TIMA Update : Outport  Port=3
  TA2 : Outport  Port=4
  wires:
  S-R Flip-Flop4/1 -> Curated Pulse Select/2, 16 * 1/f_hrtim Delay1/1  "hrtim_out_sync2 ITR10"
  HRTIM TIMA Counter/1 -> gen_tima_update/1(count), TIMA CNT/1, TIMA Count Compare to TIMD CMP1/1, "TIMA Compare 2 Op "/1, TIMA Compare 1 Op/1  "TIMA CNT"
  tima_ta2/1(ta2) -> Data Type Conversion2/1
  TIMA EEV6 Blanking/1 -> Bypass gen_tima_update/1, gen_tima_update/2(reset), HRTIM TIMA Counter/2, Rising Edge Detect1/1, Curated Pulse Select/1  "TIMA EEV6 Blanked"
  Break Algebraic Loop2/1 -> TIMA EEV8 Blanking/2
  TIMA EEV8 Blanking/1 -> tima_ta2/2(reset)  "TIMA EEV8 Blanked"
  Rising Edge Detect1/1 -> S-R Flip-Flop4/1
  TIMA Count Compare to TIMD CMP1/1 -> OR4/2
  Break Algebraic Loop/1 -> TIMA EEV9 Blanking/2
  TIMA Compare 1 Op/1 -> Break Algebraic Loop1/1  "TIMA EEV6 Blanking Source"
  16 * 1/f_hrtim Delay1/1 -> S-R Flip-Flop4/2
  OR4/1 -> tima_ta2/1(set)  "TA2 Set Src"
  Triggered Subsystem1/1(TIMA Compare 2) -> "TIMA Compare 2 Op "/2  "TIMA CMP2 Active Reg"
  No Blanking/1 -> Break Algebraic Loop2/1
  "TIMA Compare 2 Op "/1 -> Break Algebraic Loop/1, eev9_latch/2(blank_src)  "TIMA EEV9 Blank Src"
  Curated Pulse Select/1 -> hrtim_out_sync2/1
  EEV9/1 -> TIMA EEV9 Blanking/1, eev9_latch/1(eev), eev9_latch2/1(eev), NOT1/1  "EEV9"
  EEV8/1 -> TIMA EEV8 Blanking/1  "EEV8"
  EEV6/1 -> TIMA EEV6 Blanking/1  "EEV6"
  TIMD Compare 1/1 -> TIMA Count Compare to TIMD CMP1/2
  CLK/1 -> HRTIM TIMA Counter/1
  Data Type Conversion/1 -> TIMA Update/1, Triggered Subsystem2/Trigger, Triggered Subsystem1/Trigger  "TIMA Update"
  Data Type Conversion2/1 -> TA2/1  "TA2"
  Triggered Subsystem2/1(TIMA Compare 1) -> TIMA Compare 1 Op/2  "TIMA CMP1 Active Reg"
  Data Type Conversion4/1 -> Triggered Subsystem2/1(In1)
  Data Type Conversion3/1 -> Triggered Subsystem1/1(In1)
  TIMA Compare 1 Shadow Register/1 -> Data Type Conversion4/1  "TIMA CMP1"
  TIMA Compare 2 Shadow Register/1 -> Data Type Conversion3/1
  Bypass gen_tima_update/1 -> Data Type Conversion/1
  gen_tima_update/1(update) -> Bypass gen_tima_update/2
  Break Algebraic Loop1/1 -> TIMA EEV6 Blanking/2
  NOT1/1 -> Scope4/2, eev9_latch2/2(blank_src)  "Blank Src"
  eev9_latch2/1(eev_blanked) -> Scope4/3  "EEV Blanked"
  eev9_latch/1(eev_blanked) -> EEV9 Blank Latch En/2  "TIMA EEV9 Blanked"
  EEV9 Blank Latch En/1 -> OR4/1  "TIMA EEV9 Blanked"
  TIMA EEV9 Blanking/1 -> EEV9 Blank Latch En/1  "TIMA EEV9 Blanked"

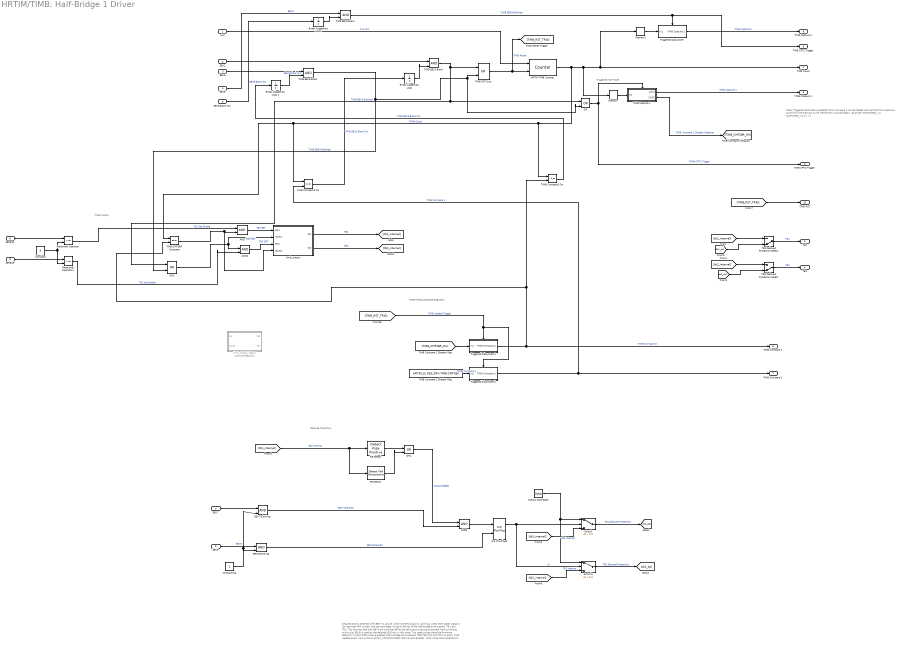
== system HRTIM/TIMB: Half-Bridge 1 Driver ==
  note: Delayed IDLE is entered when EEV7 is active (when COMP4 output is LOW,e.g. when interrupter signal is low between PRF cycles) and the next edge (rising or falling) of the Half bridge drive signals, TB1 and TB2. This ensures that the IGBTs are switched off at the next zero-crossing to prevent hard switching mid-cycle.
      |
      | EEV9 is used as the delayed IDLE exit in this case. This seeks to emulate the firmware behavior in which DMA CH5 re-enables the H-bridge drive outputs (TB1,TB2,TC1 and TC2) on every TIM5 Update event via a write to HRTIM_COMMON.OENR SFR (Output Enable). TIM5 is the interrupter/burst source and it updates every time it rolls-over (i.e. the next PRF cycle has begun).
      |
      | EEV9 is mapped to the rising edge of COMP4 output, which as mentioned, is driver by the interrupter signal.
      |
      | Thus, in this context, EEV9 event and TIM5 Update are equivalent, and thus it is used as the SR FF reset signal to "restore" the H-bridge drive signals to their enabled states.
  note: TIMB Preload Enabled Registers
  note: Triggered Half-Mode
  note: When Triggered Half-Mode is enabled: TIMx Compare 2 will be loaded with half the TIMx Capture 1 value from the previous cycle (hence the 1 sample delay). Example: COMPARE2_n = (CAPTURE1_(n-1) ) / 2
  note: TIMB Output
  note: Delayed Protection
  CLK : Inport
  EEV2 : Inport  Port=2
  EEV6 : Inport  Port=3
  EEV8 : Inport  Port=4
  EEV8 Blank Src : Inport  Port=5
  EEV9 : Inport  Port=6
  EEV7 : Inport  Port=7
  SETB1R : Inport  Port=8
  SETB2R : Inport  Port=9
  AND : Logic  IconShape=distinctive  AllPortsSameDT=off  OutDataTypeStr=boolean
  AND1 : Logic  IconShape=distinctive  AllPortsSameDT=off  OutDataTypeStr=boolean
  AND2 : Logic  IconShape=distinctive  AllPortsSameDT=off  OutDataTypeStr=boolean
  Break Algaebraic Loop : UnitDelay  SampleTime=-1  HasFrameUpgradeWarning=on
  Break Algaebraic Loop 1 : UnitDelay  SampleTime=-1  HasFrameUpgradeWarning=on
  Break Algaebraic Loop1 : UnitDelay  SampleTime=-1  HasFrameUpgradeWarning=on
  Constant : Constant  Value=0  OutDataTypeStr=uint32
  EEV7 Blanking : Logic  IconShape=distinctive  AllPortsSameDT=off  OutDataTypeStr=boolean
  EEV9 Blanking : Logic  IconShape=distinctive  AllPortsSameDT=off  OutDataTypeStr=boolean
  FE Detect : simulink/Logic and Bit Operations/Detect Fall Nonpositive  vinit=0  OutDataTypeStr=boolean
  HRTIM TIMB Counter : dspswit3/Counter  Direction=Up  CountEvent=Rising edge  CounterSize=16 bits  MaxCount=HRTIM_SL.HRTIM_TIMx_FS  InitialCount=0  Output=Count  HitValue=32  ResetInput=on  SamplesPerFrame=1  Ts=1  CntDtype=uint16  HitDtype=Logical
  Memory : Memory  InheritSampleTime=on
  Memory1 : Memory
  No Blanking : Constant
  OR : Logic  Operator=OR  IconShape=distinctive  AllPortsSameDT=off  OutDataTypeStr=boolean
  OR1 : Logic  Operator=OR  IconShape=distinctive  AllPortsSameDT=off  OutDataTypeStr=boolean
  OR2 : Logic  Operator=OR  IconShape=distinctive  AllPortsSameDT=off  OutDataTypeStr=boolean
  Output IDLE State : Constant  Value=false  OutDataTypeStr=boolean
  RE Detect : hdlsllib/Logic and Bit Operations/Detect Rise Positive  vinit=0  OutDataTypeStr=boolean
  Relational Operator : RelationalOperator  Operator=~=  OutDataTypeStr=boolean  RndMeth=Simplest  InputSameDT=off
  Relational Operator1 : RelationalOperator  Operator=~=  OutDataTypeStr=boolean  RndMeth=Simplest  InputSameDT=off
  S-R Flip-Flop6 : simulink_extras/Flip Flops/S-R Flip-Flop  initial_condition=0
  Switch : Switch  Criteria=u2 ~= 0  SaturateOnIntegerOverflow=off  InputSameDT=off
  Switch1 : Switch  Criteria=u2 ~= 0  SaturateOnIntegerOverflow=off  InputSameDT=off
  TB1 Delayed Protection Select : ManualSwitch  CurrentSetting=0
  TB2 Delayed Protection Select : ManualSwitch  CurrentSetting=0
  TIMB Capture 1 : Subsystem  TreatAsAtomicUnit=on
  TIMB Compare 1 Shadow Reg : Constant  Value=HRTIM_SL.RES_DRV.TIMB.CMP1BR
  TIMB Compare1 Op : RelationalOperator  OutDataTypeStr=boolean  RndMeth=Simplest  InputSameDT=off
  TIMB Compare2 Op : RelationalOperator  OutDataTypeStr=boolean  RndMeth=Simplest  InputSameDT=off
  TIMB EEV2 Blank : Logic  IconShape=distinctive  AllPortsSameDT=off  OutDataTypeStr=boolean
  TIMB EEV6 Blank : Logic  IconShape=distinctive  AllPortsSameDT=off  OutDataTypeStr=boolean
  TIMB EEV8 Blank : Logic  IconShape=distinctive  AllPortsSameDT=off  OutDataTypeStr=boolean
  TIMB RST Srcs : Logic  Operator=OR  IconShape=distinctive  AllPortsSameDT=off  OutDataTypeStr=boolean
  TIMB.CMP2BR Compare : RelationalOperator  Operator===  OutDataTypeStr=boolean  RndMeth=Simplest  InputSameDT=off
  Triggered Subsystem : Subsystem  TreatAsAtomicUnit=on
  Triggered Subsystem1 : Subsystem  TreatAsAtomicUnit=on
  Triggered Subsystem2 : Subsystem  TreatAsAtomicUnit=on
  timb_output : MATLAB Function  TreatAsAtomicUnit=on
  timb_output_legacy : MATLAB Function  Commented=on  TreatAsAtomicUnit=on
  TIMB Count : Outport
  TIMB CPT1 Trigger : Outport  Port=2
  TB1 : Outport  Port=3
  TB2 : Outport  Port=4
  TIMB Catpure 1 : Outport  Port=5
  TIMB Compare 2 : Outport  Port=6
  TIMB Compare 1 : Outport  Port=7
  TIMB Capture 2 : Outport  Port=8
  TIMB CPT2 Trigger : Outport  Port=9
  TIMB RST : Outport  Port=10
  wires:
  OR1/1 -> timb_output/2(reset1), AND2/1  "TB1 RST"
  TIMB EEV6 Blank/1 -> TIMB RST Srcs/2, OR/2, OR1/2  "TIMB EEV6 Blanked"
  [TIMB_CMP2BR_SH] -> Triggered Subsystem1/1(In1)
  timb_output/1(tb1) -> [tb1_internal]  "TB1"
  HRTIM TIMB Counter/1 -> Memory1/1, TIMB Count/1, Memory/1, TIMB.CMP2BR Compare/1, TIMB Compare1 Op/1, TIMB Compare2 Op/1  "TIMB Count"
  TIMB Compare1 Op/1 -> Break Algaebraic Loop/1  "TIMB EEV2 Blank Src"
  TIMB Capture 1/2(CMP2) -> [TIMB_CMP2BR_SH]  "TIMB Compare 2 Shadow Register"
  TIMB EEV2 Blank/1 -> OR/1, OR1/1, TIMB RST Srcs/1  "TIMB EEV2 Blanked"
  [TIMB_RST_TRIG] -> Triggered Subsystem2/Trigger, Triggered Subsystem1/Trigger  "TIMB Update Trigger"
  TIMB RST Srcs/1 -> HRTIM TIMB Counter/2, [TIMB_RST_TRIG]  "TIMB Reset"
  Memory/1 -> TIMB Capture 1/1(In1)
  Break Algaebraic Loop 1/1 -> TIMB EEV6 Blank/2  "EEV6 Blank Src"
  OR/1 -> TIMB CPT1 Trigger/1, TIMB Capture 1/Trigger  "TIMB CPT1 Trigger"
  Break Algaebraic Loop/1 -> TIMB EEV2 Blank/2
  Triggered Subsystem1/1(TIMB Compare 2) -> TIMB Compare2 Op/2, TIMB.CMP2BR Compare/2, TIMB Compare 2/1  "TIMB Compare 2"
  EEV2/1 -> TIMB EEV2 Blank/1
  TIMB Compare2 Op/1 -> Break Algaebraic Loop 1/1  "TIMB EEV6 Blank Src"
  Triggered Subsystem2/1(TIMB Compare 1) -> TIMB Compare1 Op/2, TIMB Compare 1/1  "TIMB Compare 1"
  TIMB Compare 1 Shadow Reg/1 -> Triggered Subsystem2/1(In1)  "TIMB Compare 1"
  TIMB Capture 1/1(CPT1) -> TIMB Catpure 1/1  "TIMB Capture 1"
  CLK/1 -> HRTIM TIMB Counter/1  "CLK Src"
  EEV6/1 -> TIMB EEV6 Blank/1
  Memory1/1 -> Triggered Subsystem/1(In1)
  Triggered Subsystem/1(TIMB Capture 2) -> TIMB Capture 2/1  "TIMB Capture 2"
  TIMB EEV8 Blank/1 -> Triggered Subsystem/Trigger, TIMB CPT2 Trigger/1  "TIMB EEV8 Blanked"
  EEV8/1 -> TIMB EEV8 Blank/1  "EEV8"
  EEV8 Blank Src/1 -> Break Algaebraic Loop1/1  "EEV8 Blank Src"
  Break Algaebraic Loop1/1 -> TIMB EEV8 Blank/2
  EEV9 Blanking/1 -> S-R Flip-Flop6/2  "EEV9 Blanked"
  S-R Flip-Flop6/1 -> Switch/2, Switch1/2  "Q"
  Output IDLE State/1 -> Switch/1, Switch1/1
  AND1/1 -> S-R Flip-Flop6/1
  FE Detect/1 -> OR2/2
  [tb1_internal] -> Switch/3  "TB1 Internal"
  OR2/1 -> AND1/1  "Output Edges"
  [tb1_internal] -> FE Detect/1, RE Detect/1  "TB1 Internal"
  RE Detect/1 -> OR2/1
  EEV7 Blanking/1 -> AND1/2  "EEV7 Blanked"
  EEV9/1 -> EEV9 Blanking/1  "EEV9"
  No Blanking/1 -> EEV9 Blanking/2, EEV7 Blanking/2
  EEV7/1 -> EEV7 Blanking/1
  timb_output/2(tb2) -> [tb2_internal]  "TB2"
  TB1 Delayed Protection Select/1 -> TB1/1  "TB1"
  TB2 Delayed Protection Select/1 -> TB2/1  "TB2"
  [tb1_internal] -> TB1 Delayed Protection Select/1
  [tb2_internal] -> TB2 Delayed Protection Select/1
  [tb2_dp] -> TB2 Delayed Protection Select/2
  [tb1_dp] -> TB1 Delayed Protection Select/2
  Switch/1 -> [tb1_dp]  "TB1 Delayed Protection"
  [tb2_internal] -> Switch1/3  "TB2 Internal"
  Switch1/1 -> [tb2_dp]  "TB2 Delayed Protection"
  [TIMB_RST_TRIG] -> TIMB RST/1
  TIMB.CMP2BR Compare/1 -> AND/2, timb_output/4(reset2)
  AND/1 -> timb_output/1(set1)  "TB1 SET"
  Constant/1 -> Relational Operator1/2, Relational Operator/2
  SETB1R/1 -> Relational Operator/1
  SETB2R/1 -> Relational Operator1/1
  Relational Operator/1 -> AND/1  "TB1 Set Enable"
  Relational Operator1/1 -> AND2/2  "TB2 Set Enable"
  AND2/1 -> timb_output/3(set2)  "TB2 SET"
